simulink model "s_b16a4x512f"  (R2016b)
settings: Solver=VariableStepDiscrete  StartTime=0.0  StopTime=1  RelTol=1e-3
undefined symbols (not defined in the file): fft_stages, n_bits_ants, n_bits_xengs
libraries: xbsIndex_r4 x23057, casper_library_misc x150, xbsReplacements_r4 x9, casper_library_delays x8, xps_library x3
(part 8 of 210)

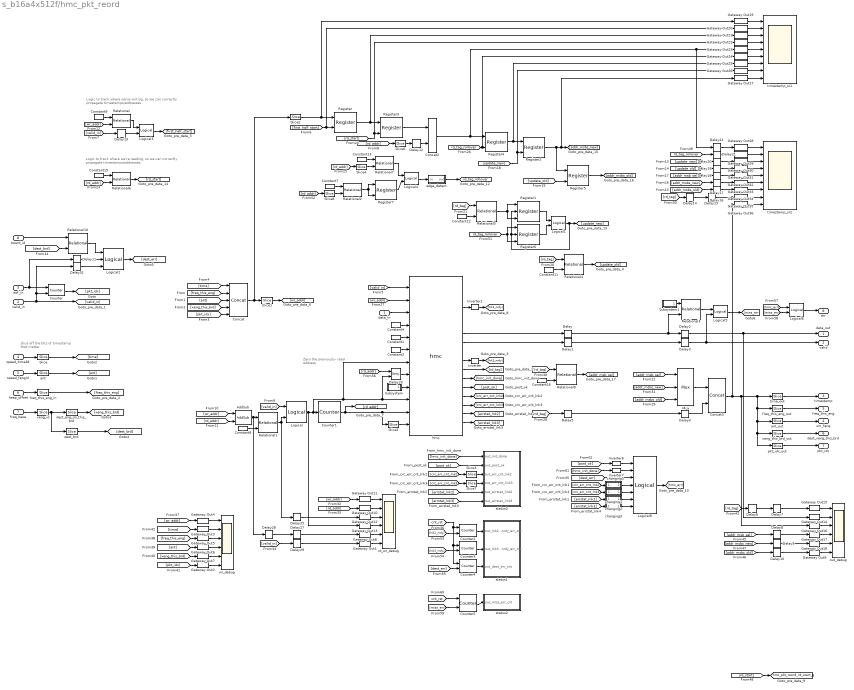
== system s_b16a4x512f/hmc_pkt_reord ==
  note: Zero the previously-
      | read address.
  note: Logic to track where we're writing,
      | so we can correctly propagate timestamps/addresses.
  note: slice off the bits of timestamp
      | that matter
  note: Logic to track where we're reading,
      | so we can correctly propagate timestamps/addresses.
  data_in : Inport
  valid_in : Inport  Port=2
  eof_in : Inport  Port=3
  spead_time48 : Inport  Port=4
  spead_fengid : Inport  Port=5
  heap_offset : Inport  Port=6
  freq_base : Inport  Port=7
  board_id : Inport  Port=8
  AddSub : xbsIndex_r4/AddSub  mode=Subtraction  use_carryin=off  use_carryout=off  en=off  latency=1  precision=User Defined  arith_type=Unsigned  n_bits=mem_depth  bin_pt=0  quantization=Truncate  overflow=Wrap  use_behavioral_HDL=off  hw_selection=Fabric  pipelined=off  dbl_ovrd=off  block_type=addsub
  Concat : xbsIndex_r4/Concat  num_inputs=5  dbl_ovrd=off  block_type=concat
  Concat2 : xbsIndex_r4/Concat  num_inputs=2  dbl_ovrd=off  block_type=concat
  Concat3 : xbsIndex_r4/Concat  num_inputs=2  dbl_ovrd=off  block_type=concat
  Constant1 : xbsIndex_r4/Constant  const=0  gui_display_data_type=Fixed-point  arith_type=Unsigned  n_bits=27  bin_pt=0  preci_type=Single  exp_width=8  frac_width=24  explicit_period=on  period=1  equ=P=C  opselect=C  inp2=PCIN>>17  opr=+  inp1=P  carry=CIN  dbl_ovrd=off  block_type=constant
  Constant11 : xbsIndex_r4/Constant  const=512*0.25  gui_display_data_type=Fixed-point  arith_type=Unsigned  n_bits=9  bin_pt=0  preci_type=Single  exp_width=8  frac_width=24  explicit_period=on  period=1  equ=P=C  opselect=C  inp2=PCIN>>17  opr=+  inp1=P  carry=CIN  dbl_ovrd=off  block_type=constant
  Constant12 : xbsIndex_r4/Constant  const=512*0.75  gui_display_data_type=Fixed-point  arith_type=Unsigned  n_bits=9  bin_pt=0  preci_type=Single  exp_width=8  frac_width=24  explicit_period=on  period=1  equ=P=C  opselect=C  inp2=PCIN>>17  opr=+  inp1=P  carry=CIN  dbl_ovrd=off  block_type=constant
  Constant13 : xbsIndex_r4/Constant  const=0  gui_display_data_type=Fixed-point  arith_type=Unsigned  n_bits=9  bin_pt=0  preci_type=Single  exp_width=8  frac_width=24  explicit_period=on  period=1  equ=P=C  opselect=C  inp2=PCIN>>17  opr=+  inp1=P  carry=CIN  dbl_ovrd=off  block_type=constant
  Constant15 : xbsIndex_r4/Constant  const=0  gui_display_data_type=Fixed-point  arith_type=Unsigned  n_bits=mem_depth  bin_pt=0  preci_type=Single  exp_width=8  frac_width=24  explicit_period=on  period=1  equ=P=C  opselect=C  inp2=PCIN>>17  opr=+  inp1=P  carry=CIN  dbl_ovrd=off  block_type=constant
  Constant16 : xbsIndex_r4/Constant  const=512*0.5  gui_display_data_type=Fixed-point  arith_type=Unsigned  n_bits=9  bin_pt=0  preci_type=Single  exp_width=8  frac_width=24  explicit_period=on  period=1  equ=P=C  opselect=C  inp2=PCIN>>17  opr=+  inp1=P  carry=CIN  dbl_ovrd=off  block_type=constant
  Constant2 : xbsIndex_r4/Constant  const=0  gui_display_data_type=Fixed-point  arith_type=Unsigned  n_bits=9  bin_pt=0  preci_type=Single  exp_width=8  frac_width=24  explicit_period=on  period=1  equ=P=C  opselect=C  inp2=PCIN>>17  opr=+  inp1=P  carry=CIN  dbl_ovrd=off  block_type=constant
  Constant4 : xbsIndex_r4/Constant  const=0  gui_display_data_type=Boolean  arith_type=Boolean  n_bits=64  bin_pt=0  preci_type=Single  exp_width=8  frac_width=24  explicit_period=on  period=1  equ=P=C  opselect=C  inp2=PCIN>>17  opr=+  inp1=P  carry=CIN  dbl_ovrd=off  block_type=constant
  Constant7 : xbsIndex_r4/Constant  const=511  gui_display_data_type=Fixed-point  arith_type=Unsigned  n_bits=9  bin_pt=0  preci_type=Single  exp_width=8  frac_width=24  explicit_period=on  period=1  equ=P=C  opselect=C  inp2=PCIN>>17  opr=+  inp1=P  carry=CIN  dbl_ovrd=off  block_type=constant
  Constant8 : xbsIndex_r4/Constant  const=2^(mem_depth-1)  gui_display_data_type=Fixed-point  arith_type=Unsigned  n_bits=mem_depth  bin_pt=0  preci_type=Single  exp_width=8  frac_width=24  explicit_period=on  period=1  equ=P=C  opselect=C  inp2=PCIN>>17  opr=+  inp1=P  carry=CIN  dbl_ovrd=off  block_type=constant
  Constant9 : xbsIndex_r4/Constant  const=2^(mem_depth)*1/4  gui_display_data_type=Fixed-point  arith_type=Unsigned  n_bits=mem_depth  bin_pt=0  preci_type=Single  exp_width=8  frac_width=24  explicit_period=on  period=1  equ=P=C  opselect=C  inp2=PCIN>>17  opr=+  inp1=P  carry=CIN  dbl_ovrd=off  block_type=constant
  Counter : xbsIndex_r4/Counter  cnt_type=Free Running  cnt_to=Inf  operation=Up  start_count=0  cnt_by_val=1  arith_type=Unsigned  n_bits=acc_bits-time_bits  bin_pt=0  load_pin=off  rst=on  en=on  explicit_period=on  period=1  use_behavioral_HDL=off  implementation=Fabric  dbl_ovrd=off  block_type=counter
  Counter1 : xbsIndex_r4/Counter  cnt_type=Free Running  cnt_to=Inf  operation=Up  start_count=0  cnt_by_val=1  arith_type=Unsigned  n_bits=mem_depth  bin_pt=0  load_pin=off  rst=off  en=on  explicit_period=on  period=1  use_behavioral_HDL=off  implementation=Fabric  dbl_ovrd=off  block_type=counter
  Counter2 : xbsIndex_r4/Counter  cnt_type=Free Running  cnt_to=Inf  operation=Up  start_count=0  cnt_by_val=1  arith_type=Unsigned  n_bits=8  bin_pt=0  load_pin=off  rst=on  en=on  explicit_period=on  period=1  use_behavioral_HDL=off  implementation=Fabric  dbl_ovrd=off  block_type=counter
  Counter3 : xbsIndex_r4/Counter  cnt_type=Free Running  cnt_to=Inf  operation=Up  start_count=0  cnt_by_val=1  arith_type=Unsigned  n_bits=8  bin_pt=0  load_pin=off  rst=on  en=on  explicit_period=on  period=1  use_behavioral_HDL=off  implementation=Fabric  dbl_ovrd=off  block_type=counter
  Counter4 : xbsIndex_r4/Counter  cnt_type=Free Running  cnt_to=Inf  operation=Up  start_count=0  cnt_by_val=1  arith_type=Unsigned  n_bits=16  bin_pt=0  load_pin=off  rst=on  en=on  explicit_period=on  period=1  use_behavioral_HDL=off  implementation=Fabric  dbl_ovrd=off  block_type=counter
  Counter5 : xbsIndex_r4/Counter  cnt_type=Free Running  cnt_to=Inf  operation=Up  start_count=0  cnt_by_val=1  arith_type=Unsigned  n_bits=32  bin_pt=0  load_pin=off  rst=on  en=on  explicit_period=on  period=1  use_behavioral_HDL=off  implementation=Fabric  dbl_ovrd=off  block_type=counter
  Delay{,1..10,12..22,25,27..29} (26 alike) : xbsIndex_r4/Delay  rst=off  infoeditControl=Selection of Reset will increase slice count due to use of real FFs and instead of SRLs  en=off  latency=1  reg_retiming=on  dbl_ovrd=off  block_type=delay
      settings: infoedit=Hardware notes: A delay line is a chain, each link of which is an SRL16 or SRL32 followed by a flip-flop.
  Delay11 : xbsIndex_r4/Delay  rst=off  infoeditControl=Selection of Reset will increase slice count due to use of real FFs and instead of SRLs  en=off  latency=2  reg_retiming=on  dbl_ovrd=off  block_type=delay
      settings: infoedit=Hardware notes: A delay line is a chain, each link of which is an SRL16 or SRL32 followed by a flip-flop.
  Delay23 : xbsIndex_r4/Delay  rst=off  infoeditControl=Selection of Reset will increase slice count due to use of real FFs and instead of SRLs  en=on  latency=62  reg_retiming=off  dbl_ovrd=off  block_type=delay
      settings: infoedit=Hardware notes: A delay line is a chain, each link of which is an SRL16 or SRL32 followed by a flip-flop.
  Delay31 : xbsIndex_r4/Delay  rst=off  infoeditControl=Selection of Reset will increase slice count due to use of real FFs and instead of SRLs  en=off  latency=2  reg_retiming=on  dbl_ovrd=off  block_type=delay
      settings: infoedit=Hardware notes: A delay line is a chain, each link of which is an SRL16 or SRL32 followed by a flip-flop.
  Gateway Out{1..18} (18 alike) : xbsIndex_r4/Gateway Out  inherit_from_input=off  hdl_port=off  rows=1  columns=1  UseAsDAC=off  DACChannel='1'  interface=None  automatic_assignment=on  address_offset=hex2dec('00')  intf_name=''  intf_description=''  timing_constraint=None  locs_specified=off  LOCs={}  io_standard={}  block_type=gatewayout
      settings: infoedit="Gateway out block.  Converts Xilinx fixed point inputs into ouputs of type Simulink integer, double, or fixed point.<P><P>Hardware notes:  In hardware these blocks become top level output ports or are discarded, depending on how they are configured."  xl_area=[0, 0, 0, 0, 0, 0, 0]  block_version=10.1.3
  Gateway Out{19..36} (18 alike) : xbsIndex_r4/Gateway Out  inherit_from_input=off  hdl_port=on  rows=1  columns=1  UseAsDAC=off  DACChannel='1'  interface=None  automatic_assignment=on  address_offset=hex2dec('00')  intf_name=''  intf_description=''  timing_constraint=None  locs_specified=off  LOCs={}  io_standard={}  block_type=gatewayout
  Inverter{,1,6..7} (4 alike) : xbsIndex_r4/Inverter  en=off  latency=0  dbl_ovrd=off  block_type=inv
  Logical : xbsIndex_r4/Logical  logical_function=AND  inputs=2  en=off  latency=1  precision=Full  arith_type=Unsigned  n_bits=16  bin_pt=0  align_bp=on  dbl_ovrd=off  block_type=logical
  Logical{1,3..5} (4 alike) : xbsIndex_r4/Logical  logical_function=AND  inputs=2  en=off  latency=0  precision=Full  arith_type=Unsigned  n_bits=16  bin_pt=0  align_bp=on  dbl_ovrd=off  block_type=logical
  Logical2 : xbsIndex_r4/Logical  logical_function=AND  inputs=3  en=off  latency=1  precision=Full  arith_type=Unsigned  n_bits=16  bin_pt=0  align_bp=on  dbl_ovrd=off  block_type=logical
  Logical6 : xbsIndex_r4/Logical  logical_function=OR  inputs=2  en=off  latency=0  precision=Full  arith_type=Unsigned  n_bits=16  bin_pt=0  align_bp=on  dbl_ovrd=off  block_type=logical
  Logical9 : xbsIndex_r4/Logical  logical_function=OR  inputs=7  en=off  latency=1  precision=Full  arith_type=Unsigned  n_bits=16  bin_pt=0  align_bp=on  dbl_ovrd=off  block_type=logical
  Mux : xbsIndex_r4/Mux  inputs=2  en=off  latency=1  precision=Full  arith_type=Unsigned  n_bits=16  bin_pt=14  quantization=Truncate  overflow=Wrap  dbl_ovrd=off  block_type=mux
  Register{,2..5,7} (6 alike) : xbsIndex_r4/Register  init=0  rst=off  en=on  dbl_ovrd=off  block_type=register
  Register1 : xbsIndex_r4/Register  init=0  rst=on  en=on  dbl_ovrd=off  block_type=register
  Register6 : xbsIndex_r4/Register  init=0  rst=on  en=on  dbl_ovrd=off  block_type=register
  Relational : xbsIndex_r4/Relational  mode=a>=b  op_type=Bool  en=off  latency=1  dbl_ovrd=off  block_type=relational
  Relational1 : xbsIndex_r4/Relational  mode=a>=b  op_type=Bool  en=off  latency=1  dbl_ovrd=off  block_type=relational
  Relational10 : xbsIndex_r4/Relational  mode=a!=b  op_type=Bool  en=off  latency=2  dbl_ovrd=off  block_type=relational
  Relational{2..3,6..7} (4 alike) : xbsIndex_r4/Relational  mode=a=b  op_type=Bool  en=off  latency=1  dbl_ovrd=off  block_type=relational
  Relational4 : xbsIndex_r4/Relational  mode=a=b  op_type=Bool  en=off  latency=0  dbl_ovrd=off  block_type=relational
  Relational5 : xbsIndex_r4/Relational  mode=a=b  op_type=Bool  en=off  latency=0  dbl_ovrd=off  block_type=relational
  Relational9 : xbsIndex_r4/Relational  mode=a>b  op_type=Bool  en=off  latency=1  dbl_ovrd=off  block_type=relational
  Slice : xbsIndex_r4/Slice  nbits=1  boolean_output=off  mode=Two Bit Locations  bit1=0  base1=MSB of Input  bit0=(freq_bits+1) + acc_bits  base0=LSB of Input  dbl_ovrd=off  block_type=slice
  Slice1 : xbsIndex_r4/Slice  nbits=mem_depth  boolean_output=off  mode=Lower Bit Location + Width  bit1=0  base1=MSB of Input  bit0=0  base0=LSB of Input  dbl_ovrd=off  block_type=slice
  Slice2 : xbsIndex_r4/Slice  nbits=27  boolean_output=off  mode=Two Bit Locations  bit1=0  base1=MSB of Input  bit0=mem_depth  base0=LSB of Input  dbl_ovrd=off  block_type=slice
  Slice3 : xbsIndex_r4/Slice  nbits=8  boolean_output=off  mode=Lower Bit Location + Width  bit1=0  base1=MSB of Input  bit0=0  base0=LSB of Input  dbl_ovrd=off  block_type=slice
  Slice4 : xbsIndex_r4/Slice  nbits=9  boolean_output=off  mode=Lower Bit Location + Width  bit1=0  base1=MSB of Input  bit0=0  base0=LSB of Input  dbl_ovrd=off  block_type=slice
  Slice5 : xbsIndex_r4/Slice  nbits=9  boolean_output=off  mode=Lower Bit Location + Width  bit1=0  base1=MSB of Input  bit0=0  base0=LSB of Input  dbl_ovrd=off  block_type=slice
  Slice6 : xbsIndex_r4/Slice  nbits=mem_depth  boolean_output=off  mode=Two Bit Locations  bit1=0  base1=MSB of Input  bit0=9  base0=LSB of Input  dbl_ovrd=off  block_type=slice
  Slice7 : xbsIndex_r4/Slice  nbits=8  boolean_output=off  mode=Lower Bit Location + Width  bit1=0  base1=MSB of Input  bit0=0  base0=LSB of Input  dbl_ovrd=off  block_type=slice
  Slice8 : xbsIndex_r4/Slice  nbits=9  boolean_output=off  mode=Lower Bit Location + Width  bit1=0  base1=MSB of Input  bit0=0  base0=LSB of Input  dbl_ovrd=off  block_type=slice
  Subsystem : Subsystem
  Subsystem1 : Subsystem
  ant : xbsIndex_r4/Slice  nbits=ant_bits  boolean_output=off  mode=Lower Bit Location + Width  bit1=0  base1=MSB of Input  bit0=0  base0=LSB of Input  dbl_ovrd=off  block_type=slice
      settings: block_version=10.1.3
  ant_out : xbsIndex_r4/Slice  nbits=ant_bits  boolean_output=off  mode=Lower Bit Location + Width  bit1=0  base1=MSB of Input  bit0=acc_bits+share_bits-time_bits  base0=LSB of Input  dbl_ovrd=off  block_type=slice
      settings: block_version=10.1.3
  changing0 : Subsystem
  changing1 : Subsystem
  changing2 : Subsystem
  changing3 : Subsystem
  dest_brd : xbsIndex_r4/Slice  nbits=xeng_bits-share_bits  boolean_output=off  mode=Upper Bit Location + Width  bit1=0  base1=MSB of Input  bit0=freq_bits-xeng_bits  base0=LSB of Input  dbl_ovrd=off  block_type=slice
      settings: block_version=10.1.3
  dest_eng_on_this_brd : xbsIndex_r4/Slice  nbits=share_bits  boolean_output=off  mode=Lower Bit Location + Width  bit1=0  base1=MSB of Input  bit0=0  base0=LSB of Input  dbl_ovrd=off  block_type=slice
      settings: block_version=10.1.3
  edge_detect : Subsystem  AncestorBlock=casper_library_misc/edge_detect  mask(edge_detect){edge=Falling, polarity=Active High, x_in=[0 0.08 0.08 0.16 0.16 0.24 0.24 0.32 0.32 0.4], y_in=[-1 -1  1  1  1  1  1  1  1  1], x_out=[0.6 0.68 0.68 0.76 0.76 0.84 0.84 0.92 0.92 1], y_out=[-1 -1  1  1 -1 -1 -1 -1 -1 -1]}
      mask prompts: edge "Edge Type"; polarity "Output Polarity"; x_in "Input X Positions"; y_in "Input Y Positions"; x_out "Output X Positions"; y_out "Output Y Positions"
      mask help: Output is active for one-cycle after each edge of the specified type (i.e. rising, falling or both).
      mask init: same as s_b16a4x512f/edge_detect
      settings: AttributesFormatString=|
      | falling edges
      | active high
      mask Help: Output is active for one-cycle after each edge of the specified type (i.e. rising, falling, or both).  Latency is zero.
      mask TypeOptions edge: Rising | Falling | Both
      mask TypeOptions polarity: Active High | Active Low
      mask Display:
      | plot(x_in_num,0.5+y_in_num*0.2);
      | plot(x_out_num,0.5+y_out_num*0.2);
  freq_this_eng_in : xbsIndex_r4/Slice  nbits=freq_bits - xeng_bits  boolean_output=off  mode=Lower Bit Location + Width  bit1=0  base1=LSB of Input  bit0=acc_bits-1+3  base0=LSB of Input  dbl_ovrd=off  block_type=slice
      settings: block_version=10.1.3
  freq_this_eng_out : xbsIndex_r4/Slice  nbits=freq_bits - xeng_bits  boolean_output=off  mode=Lower Bit Location + Width  bit1=0  base1=LSB of Input  bit0=acc_bits+share_bits+ant_bits-time_bits  base0=LSB of Input  dbl_ovrd=off  block_type=slice
      settings: block_version=10.1.3
  hmc : xps_library/hmc  Tag=xps:hmc  mez=2  sim_depth=12  sim_latency=10  sim_rand=on
      link override sim_mem1: randread=off
      link override sim_mem2/sfunc: depth_bits=12
  out_debug : Scope  NumInputPorts=6
  pkt_idx_out : xbsIndex_r4/Slice  nbits=acc_bits-time_bits  boolean_output=off  mode=Lower Bit Location + Width  bit1=freq_bits  base1=LSB of Input  bit0=0  base0=LSB of Input  dbl_ovrd=off  block_type=slice
      settings: block_version=10.1.3
  rd_wr_debug : Scope  NumInputPorts=6
  status0 : Subsystem  Tag=xps:sw_reg  AncestorBlock=xps_library/software_register  mask(swreg){io_dir=To Processor, io_delay=0, sample_period=1, names=[init_done post_ok err_cnt_lnk2 err_cnt_link3 errstat_link2 errstat_link3], bitwidths=[1 1 8 8 7 7], bin_pts=0, arith_types=[2 2 0 0 0 0], sim_port=off, show_format=on}
      mask prompts: io_dir "I/O direction"; io_delay "I/O delay"; sample_period "Sample period"; names "Bitfield names [msb...lsb]"; bitwidths "Bitfield widths"; bin_pts "Bitfield binary pts"; arith_types "Bitfield types, ufix=0, fix=1, bool=2"; sim_port "Provide sim input/output?"; show_format "Print format string?"
      mask help: A 32-bit software-accessible register. Can be divided into bitfields of varying widths and types using the fields in the block mask.
      mask init:
      | swreg_init(gcb)
      settings: AttributesFormatString=6 outputs:b,b,uf8.0,uf8.0,uf7.0,uf7.0 = 32 bits
      mask TypeOptions io_dir: To Processor | From Processor
      mask Callback io_dir:
      | mask_enables = get_param(gcb, 'MaskEnables');
      | mask_names = get_param(gcb, 'MaskNames');
      | if strcmp(get_param(gcb, 'io_dir'), 'To Processor'),
      |     mask_enables{ismember(mask_names, 'sample_period')} = 'off';
      | else
      |     mask_enables{ismember(mask_names, 'sample_period')} = 'on';
      | end
      | set_param(gcb, 'MaskEnables', mask_enables);
  status1 : Subsystem  Tag=xps:sw_reg  AncestorBlock=xps_library/software_register  mask(swreg){io_dir=To Processor, io_delay=0, sample_period=1, names=[lnk2_nrdy_err_cnt lnk3_nrdy_err_cnt dest_err_cnt], bitwidths=[8 8 16], bin_pts=0, arith_types=0, sim_port=off, show_format=on}
      mask prompts: io_dir "I/O direction"; io_delay "I/O delay"; sample_period "Sample period"; names "Bitfield names [msb...lsb]"; bitwidths "Bitfield widths"; bin_pts "Bitfield binary pts"; arith_types "Bitfield types, ufix=0, fix=1, bool=2"; sim_port "Provide sim input/output?"; show_format "Print format string?"
      mask help: A 32-bit software-accessible register. Can be divided into bitfields of varying widths and types using the fields in the block mask.
      mask init:
      | swreg_init(gcb)
      settings: AttributesFormatString=3 outputs:uf8.0,uf8.0,uf16.0 = 32 bits
      mask TypeOptions io_dir: To Processor | From Processor
      mask Callback io_dir:
      | mask_enables = get_param(gcb, 'MaskEnables');
      | mask_names = get_param(gcb, 'MaskNames');
      | if strcmp(get_param(gcb, 'io_dir'), 'To Processor'),
      |     mask_enables{ismember(mask_names, 'sample_period')} = 'off';
      | else
      |     mask_enables{ismember(mask_names, 'sample_period')} = 'on';
      | end
      | set_param(gcb, 'MaskEnables', mask_enables);
  status2 : Subsystem  Tag=xps:sw_reg  AncestorBlock=xps_library/software_register  mask(swreg){io_dir=To Processor, io_delay=0, sample_period=1, names=[miss_err_cnt], bitwidths=[32], bin_pts=0, arith_types=0, sim_port=off, show_format=on}
      mask prompts: io_dir "I/O direction"; io_delay "I/O delay"; sample_period "Sample period"; names "Bitfield names [msb...lsb]"; bitwidths "Bitfield widths"; bin_pts "Bitfield binary pts"; arith_types "Bitfield types, ufix=0, fix=1, bool=2"; sim_port "Provide sim input/output?"; show_format "Print format string?"
      mask help: A 32-bit software-accessible register. Can be divided into bitfields of varying widths and types using the fields in the block mask.
      mask init:
      | swreg_init(gcb)
      settings: AttributesFormatString=1output:uf32.0 = 32 bits
      mask TypeOptions io_dir: To Processor | From Processor
      mask Callback io_dir:
      | mask_enables = get_param(gcb, 'MaskEnables');
      | mask_names = get_param(gcb, 'MaskNames');
      | if strcmp(get_param(gcb, 'io_dir'), 'To Processor'),
      |     mask_enables{ismember(mask_names, 'sample_period')} = 'off';
      | else
      |     mask_enables{ismember(mask_names, 'sample_period')} = 'on';
      | end
      | set_param(gcb, 'MaskEnables', mask_enables);
  time_out : xbsIndex_r4/Slice  nbits=1  boolean_output=off  mode=Two Bit Locations  bit1=0  base1=MSB of Input  bit0=acc_bits+share_bits+ant_bits+freq_bits-xeng_bits-time_bits  base0=LSB of Input  dbl_ovrd=off  block_type=slice
  timestamp_sr1 : Scope  NumInputPorts=9
  timestamp_sr2 : Scope  NumInputPorts=9
  wr_debug : Scope  NumInputPorts=6
  xeng_id : xbsIndex_r4/Slice  nbits=xeng_bits  boolean_output=off  mode=Lower Bit Location + Width  bit1=freq_bits  base1=LSB of Input  bit0=freq_bits-xeng_bits  base0=LSB of Input  dbl_ovrd=off  block_type=slice
      settings: block_version=10.1.3
  xeng_this_brd_out : xbsIndex_r4/Slice  nbits=share_bits  boolean_output=off  mode=Lower Bit Location + Width  bit1=freq_bits  base1=LSB of Input  bit0=acc_bits-time_bits  base0=LSB of Input  dbl_ovrd=off  block_type=slice
      settings: block_version=10.1.3
  data_out : Outport
  valid : Outport  Port=2
  timestamp : Outport  Port=3
  src_feng : Outport  Port=4
  freq_this_eng : Outport  Port=5
  dest_xeng_this_brd : Outport  Port=6
  pkt_idx : Outport  Port=7
  err : Outport  Port=8
  tag scope: hmc_pkt_reord_rd_start_g=global, rd_tag_rollover=global
  wires:
  Gateway Out1/1 -> rd_wr_debug/6
  Gateway Out10/1 -> rd_wr_debug/2
  Gateway Out11/1 -> rd_wr_debug/1
  Gateway Out12/1 -> rd_wr_debug/3
  Gateway Out13/1 -> rd_wr_debug/4
  Gateway Out8/1 -> rd_wr_debug/5
  heap_offset/1 -> freq_this_eng_in/1
  xeng_id/1 -> dest_eng_on_this_brd/1, dest_brd/1
  spead_fengid/1 -> ant/1
  spead_time48/1 -> Slice/1
  freq_base/1 -> xeng_id/1
  [xeng_this_brd] -> Concat/4
  [pkt_idx] -> Concat/5
  [freq_this_eng] -> Concat/2
  [ant] -> Concat/3
  [time] -> Concat/1
  Concat/1 -> Slice2/1, Slice1/1
  data_in/1 -> hmc/3
  eof_in/1 -> Counter/1, Delay11/1
  valid_in/1 -> [valid_in], Delay31/1, Counter/2
  [valid_in] -> hmc/1
  Counter/1 -> [pkt_idx]
  ant/1 -> [ant]
  Slice/1 -> [time]
  dest_eng_on_this_brd/1 -> [xeng_this_brd]
  freq_this_eng_in/1 -> [freq_this_eng]
  Delay23/1 -> hmc/8
  Subsystem/1(Out1) -> hmc/9
  [first_half_start] -> Gateway Out20/1, Register/2
  Slice2/1 -> Gateway Out19/1, Register/1
  Counter1/1 -> hmc/11, Slice5/1, [rd_addr]
  Slice5/1 -> hmc/12
  [valid_in] -> Logical/1
  Constant8/1 -> Relational1/2
  AddSub/1 -> Delay28/1, Relational1/1
  [wr_addr] -> AddSub/1
  [rd_addr] -> AddSub/2
  Relational1/1 -> Delay25/1, Logical/2
  Constant9/1 -> Relational/1
  [wr_addr] -> Relational/2
  [rd_tag] -> Relational4/1
  Constant11/1 -> Relational4/2
  Constant12/1 -> Relational5/2
  [rd_tag] -> Relational5/1
  Constant15/1 -> Relational6/1
  [rd_addr] -> Relational6/2
  Relational6/1 -> [rd_start]
  Register/1 -> Gateway Out21/1, Register3/1
  [rd_start] -> Gateway Out22/1, Register3/2
  Constant13/1 -> Relational7/1
  [rd_addr] -> Slice4/1
  Slice4/1 -> Relational7/2
  Slice1/1 -> [wr_addr]
  [wr_addr] -> hmc/2
  [rd_tag_rollover] -> Gateway Out24/1, Register4/2
  Register3/1 -> Concat2/1
  Slice6/1 -> Delay12/1
  [rd_addr] -> Slice6/1
  Concat2/1 -> Gateway Out23/1, Delay22/1, Register4/1
  Relational4/1 -> [update_old]
  [rd_tag] -> Delay5/1
  Register4/1 -> Gateway Out25/1, Register2/1
  Register2/1 -> Gateway Out27/1, [addr_msbs_new], Register5/1
  [update_old] -> Register5/2
  Register5/1 -> [addr_msbs_old]
  Constant16/1 -> Relational9/2
  [rd_tag] -> Relational9/1
  Relational9/1 -> [addr_msb_sel]
  Mux/1 -> Concat3/1
  [addr_msb_sel] -> Mux/1
  [addr_msbs_old] -> Mux/3
  [addr_msbs_new] -> Mux/2
  Concat3/1 -> Gateway Out36/1, Gateway Out16/1, pkt_idx_out/1, xeng_this_brd_out/1, ant_out/1, freq_this_eng_out/1, time_out/1
  time_out/1 -> timestamp/1
  freq_this_eng_out/1 -> freq_this_eng/1
  ant_out/1 -> src_feng/1
  xeng_this_brd_out/1 -> dest_xeng_this_brd/1
  pkt_idx_out/1 -> pkt_idx/1
  Delay/1 -> Relational3/2, Delay2/1
  Delay1/1 -> Delay3/1
  Delay2/1 -> data_out/1, Gateway Out14/1
  Delay4/1 -> Concat3/2
  Delay5/1 -> Delay4/1
  [wr_addr] -> Gateway Out11/1
  [rd_addr] -> Gateway Out10/1
  dest_brd/1 -> [dest_brd]
  Gateway Out2/1 -> wr_debug/6
  Gateway Out3/1 -> wr_debug/2
  Gateway Out4/1 -> wr_debug/1
  Gateway Out5/1 -> wr_debug/3
  Gateway Out6/1 -> wr_debug/4
  Gateway Out7/1 -> wr_debug/5
  [wr_addr] -> Gateway Out4/1
  [time] -> Gateway Out3/1
  [freq_this_eng] -> Gateway Out5/1
  [ant] -> Gateway Out6/1
  [xeng_this_brd] -> Gateway Out7/1
  [pkt_idx] -> Gateway Out2/1
  Gateway Out9/1 -> out_debug/6
  Gateway Out14/1 -> out_debug/2
  Gateway Out15/1 -> out_debug/1
  Gateway Out16/1 -> out_debug/3
  Gateway Out17/1 -> out_debug/4
  Gateway Out18/1 -> out_debug/5
  [addr_msb_sel] -> Delay8/1
  [addr_msbs_new] -> Delay9/1
  [addr_msbs_old] -> Delay10/1
  [rd_tag] -> Delay6/1
  Delay6/1 -> Delay7/1
  Delay7/1 -> Gateway Out15/1
  Delay8/1 -> Gateway Out17/1
  Delay9/1 -> Gateway Out18/1
  Delay10/1 -> Gateway Out9/1
  Slice3/1 -> status0/3(out_err_cnt_lnk2)
  Slice7/1 -> status0/4(out_err_cnt_link3)
  [dest_brd] -> Relational10/2
  board_id/1 -> Relational10/1
  Relational10/1 -> Logical2/1
  Delay11/1 -> Logical2/2
  Gateway Out23/1 -> timestamp_sr1/5
  Gateway Out26/1 -> timestamp_sr1/8
  Gateway Out20/1 -> timestamp_sr1/2
  Gateway Out19/1 -> timestamp_sr1/1
  Gateway Out25/1 -> timestamp_sr1/7
  Gateway Out22/1 -> timestamp_sr1/4
  Gateway Out21/1 -> timestamp_sr1/3
  Gateway Out24/1 -> timestamp_sr1/6
  Gateway Out27/1 -> timestamp_sr1/9
  [update_new] -> Gateway Out26/1, Register2/2
  Delay12/1 -> Concat2/2
  Logical3/1 -> [first_half_start]
  Relational/1 -> Logical3/1
  [valid_in] -> Delay13/1
  Delay13/1 -> Logical3/2
  Gateway Out32/1 -> timestamp_sr2/5
  Gateway Out35/1 -> timestamp_sr2/8
  Gateway Out29/1 -> timestamp_sr2/2
  Gateway Out28/1 -> timestamp_sr2/1
  Gateway Out34/1 -> timestamp_sr2/7
  Gateway Out31/1 -> timestamp_sr2/4
  Gateway Out30/1 -> timestamp_sr2/3
  Gateway Out33/1 -> timestamp_sr2/6
  Gateway Out36/1 -> timestamp_sr2/9
  [rd_tag_rollover] -> Delay21/1
  [update_new] -> Delay20/1
  [update_old] -> Delay19/1
  [addr_msb_sel] -> Delay18/1
  [addr_msbs_new] -> Delay17/1
  [addr_msbs_old] -> Delay16/1
  [rd_tag] -> Delay14/1
  Delay14/1 -> Delay15/1
  Delay15/1 -> Gateway Out35/1
  Delay16/1 -> Gateway Out34/1
  Delay17/1 -> Gateway Out33/1
  Delay18/1 -> Gateway Out32/1
  Delay19/1 -> Gateway Out31/1
  Delay20/1 -> Gateway Out30/1
  Delay21/1 -> Gateway Out29/1
  Delay22/1 -> Gateway Out28/1
  Relational5/1 -> Register1/3, Register1/1
  [rd_tag_rollover] -> Register6/1, Register6/3
  Register1/1 -> Logical1/1
  Register6/1 -> Logical1/2
  Logical1/1 -> Register6/2, Register1/2, [update_new]
  Relational7/1 -> Logical4/1
  Register7/1 -> Logical4/2
  Constant7/1 -> Relational2/1
  [rd_addr] -> Slice8/1
  Slice8/1 -> Relational2/2
  Relational2/1 -> Register7/2, Register7/1
  Logical4/1 -> edge_detect/1(in)
  edge_detect/1(out) -> [rd_tag_rollover]
  [valid_in] -> Delay29/1
  Delay25/1 -> Gateway Out12/1
  Delay27/1 -> Gateway Out8/1
  Delay28/1 -> Delay27/1
  Delay29/1 -> Gateway Out1/1
  Subsystem1/1(Out1) -> Relational3/1
  Relational3/1 -> Logical5/1
  Delay3/1 -> Logical5/2, valid/1
  Logical2/1 -> [dest_err]
  Logical6/1 -> err/1
  [cnt_rst] -> Counter4/1, Counter3/1, Counter2/1
  Counter2/1 -> status1/1(out_lnk2_nrdy_err_cnt)
  Counter3/1 -> status1/2(out_lnk3_nrdy_err_cnt)
  Counter4/1 -> status1/3(out_dest_err_cnt)
  hmc/9 -> Inverter/1
  Inverter/1 -> [lnk3_nrdy]
  hmc/3 -> Inverter1/1
  Inverter1/1 -> [lnk2_nrdy]
  [dest_err] -> Counter4/2
  [lnk2_nrdy] -> Counter2/2
  [lnk3_nrdy] -> Counter3/2
  Logical/1 -> Gateway Out13/1, Delay23/2, hmc/10, hmc/7, Counter1/1
  Delay31/1 -> Logical2/3
  [rd_start] -> [hmc_pkt_reord_rd_start_g]
  Constant2/1 -> hmc/6
  Constant1/1 -> hmc/5
  Constant4/1 -> hmc/4
  hmc/10 -> [rd_tag]
  hmc/6 -> Delay/1
  hmc/7 -> Delay1/1
  [post_ok] -> Inverter6/1
  Inverter6/1 -> Logical9/1
  [hmc_init_done] -> Inverter7/1
  hmc/11 -> [hmc_init_done]
  hmc/12 -> [post_ok]
  hmc/13 -> [crc_err_cnt_lnk2]
  hmc/14 -> [crc_err_cnt_lnk3]
  hmc/15 -> [errstat_lnk2]
  hmc/16 -> [errstat_lnk3]
  [post_ok] -> status0/2(out_post_ok)
  [hmc_init_done] -> status0/1(out_init_done)
  [crc_err_cnt_lnk2] -> Slice3/1
  [crc_err_cnt_lnk3] -> Slice7/1
  [errstat_lnk2] -> status0/5(out_errstat_link2)
  [errstat_lnk3] -> status0/6(out_errstat_link3)
  Inverter7/1 -> Logical9/2
  [dest_err] -> Logical9/3
  [crc_err_cnt_lnk2] -> changing0/1(In1)
  changing0/1(Out1) -> Logical9/4
  changing3/1(Out1) -> Logical9/7
  changing1/1(Out1) -> Logical9/5
  changing2/1(Out1) -> Logical9/6
  [crc_err_cnt_lnk3] -> changing1/1(In1)
  [errstat_lnk2] -> changing2/1(In1)
  [errstat_lnk3] -> changing3/1(In1)
  Logical9/1 -> [hmc_err]
  [hmc_err] -> Logical6/1
  [rd_addr] -> Delay23/1
  [miss_err] -> Logical6/2
  Logical5/1 -> [miss_err]
  [miss_err] -> Counter5/2
  [cnt_rst] -> Counter5/1
  Counter5/1 -> status2/1(out_miss_err_cnt)

== system s_b16a4x512f/hmc_pkt_reord_status ==
  out_err_cnt : Inport
  assert_err_cnt : xbsIndex_r4/Assert  assert_type=on  type_source=Explicitly  gui_display_data_type=Fixed-point  arith_type=Unsigned  n_bits=32  bin_pt=0  preci_type=Single  exp_width=8  frac_width=24  assert_rate=off  rate_source=Explicitly  period=1  output_port=on  block_type=assert
  cast_gw : xbsIndex_r4/Convert  gui_display_data_type=Fixed-point  arith_type=Unsigned  n_bits=32  bin_pt=0  float_type=Single  exp_bits=8  fraction_bits=24  quantization=Truncate  overflow=Wrap  en=off  latency=1  pipeline=off  dbl_ovrd=off  block_type=convert
  io_delay : xbsIndex_r4/Delay  rst=off  infoeditControl=Selection of Reset will increase slice count due to use of real FFs and instead of SRLs  en=off  latency=0  reg_retiming=on  dbl_ovrd=off  block_type=delay
      settings: infoedit=Hardware notes: A delay line is a chain, each link of which is an SRL16 or SRL32 followed by a flip-flop.
  reint1 : xbsIndex_r4/Reinterpret  force_arith_type=on  arith_type=Unsigned  force_bin_pt=on  bin_pt=0  block_type=reinterpret
  s_b16a4x512f_hmc_pkt_reord_status_user_data_in : xbsIndex_r4/Gateway Out  inherit_from_input=off  hdl_port=on  rows=1  columns=1  UseAsDAC=off  DACChannel='1'  interface=None  automatic_assignment=on  address_offset=hex2dec('00')  intf_name=''  intf_description=''  timing_constraint=None  locs_specified=off  LOCs={}  io_standard={}  block_type=gatewayout
  sim_out : Terminator
  wires:
  io_delay/1 -> cast_gw/1
  cast_gw/1 -> s_b16a4x512f_hmc_pkt_reord_status_user_data_in/1
  s_b16a4x512f_hmc_pkt_reord_status_user_data_in/1 -> sim_out/1
  out_err_cnt/1 -> assert_err_cnt/1
  assert_err_cnt/1 -> reint1/1
  reint1/1 -> io_delay/1

== system s_b16a4x512f/miss_cnt0 ==
  Convert : xbsIndex_r4/Convert  gui_display_data_type=Fixed-point  arith_type=Unsigned  n_bits=6  bin_pt=0  float_type=Single  exp_bits=8  fraction_bits=24  quantization=Truncate  overflow=Wrap  en=off  latency=0  pipeline=off  dbl_ovrd=off  block_type=convert
  Counter1 : xbsIndex_r4/Counter  cnt_type=Free Running  cnt_to=1023  operation=Up  start_count=0  cnt_by_val=1  arith_type=Unsigned  n_bits=6  bin_pt=0  load_pin=off  rst=on  en=on  explicit_period=on  period=1  use_behavioral_HDL=on  implementation=Fabric  use_rpm=on  dbl_ovrd=off  block_type=counter
      settings: xl_area=[0, 0, 0, 0, 0, 0, 0]
  Delay1 : Subsystem  AncestorBlock=casper_library_delays/pipeline  mask(pipeline){latency=2}
      mask help:
      | An explicitly laid-out delay line to avoid mapping to SRL16s
      | for use in pipelining to help achieve timing closure.
      mask init:
      | pipeline_init(gcb,'latency',latency);
      settings: AttributesFormatString=Latency = %<latency>
      mask Display:
      | port_label('input', 1, 'd');
      | port_label('output', 1, 'q');
      | disp(['Z^-', num2str(latency)]);
  Delay11 : Subsystem  AncestorBlock=casper_library_delays/pipeline  mask(pipeline){latency=2}
      mask help:
      | An explicitly laid-out delay line to avoid mapping to SRL16s
      | for use in pipelining to help achieve timing closure.
      mask init:
      | pipeline_init(gcb,'latency',latency);
      settings: AttributesFormatString=Latency = %<latency>
      mask Display:
      | port_label('input', 1, 'd');
      | port_label('output', 1, 'q');
      | disp(['Z^-', num2str(latency)]);
  Delay15 : Subsystem  AncestorBlock=casper_library_delays/pipeline  mask(pipeline){latency=2}
      mask help:
      | An explicitly laid-out delay line to avoid mapping to SRL16s
      | for use in pipelining to help achieve timing closure.
      mask init:
      | pipeline_init(gcb,'latency',latency);
      settings: AttributesFormatString=Latency = %<latency>
      mask Display:
      | port_label('input', 1, 'd');
      | port_label('output', 1, 'q');
      | disp(['Z^-', num2str(latency)]);
  Delay2 : Subsystem  AncestorBlock=casper_library_delays/pipeline  mask(pipeline){latency=2}
      mask help:
      | An explicitly laid-out delay line to avoid mapping to SRL16s
      | for use in pipelining to help achieve timing closure.
      mask init:
      | pipeline_init(gcb,'latency',latency);
      settings: AttributesFormatString=Latency = %<latency>
      mask Display:
      | port_label('input', 1, 'd');
      | port_label('output', 1, 'q');
      | disp(['Z^-', num2str(latency)]);
  Delay3 : Subsystem  AncestorBlock=casper_library_delays/pipeline  mask(pipeline){latency=2}
      mask help:
      | An explicitly laid-out delay line to avoid mapping to SRL16s
      | for use in pipelining to help achieve timing closure.
      mask init:
      | pipeline_init(gcb,'latency',latency);
      settings: AttributesFormatString=Latency = %<latency>
      mask Display:
      | port_label('input', 1, 'd');
      | port_label('output', 1, 'q');
      | disp(['Z^-', num2str(latency)]);
  Delay4 : Subsystem  AncestorBlock=casper_library_delays/pipeline  mask(pipeline){latency=1}
      mask help:
      | An explicitly laid-out delay line to avoid mapping to SRL16s
      | for use in pipelining to help achieve timing closure.
      mask init:
      | pipeline_init(gcb,'latency',latency);
      settings: AttributesFormatString=Latency = %<latency>
      mask Display:
      | port_label('input', 1, 'd');
      | port_label('output', 1, 'q');
      | disp(['Z^-', num2str(latency)]);
  Delay5 : Subsystem  AncestorBlock=casper_library_delays/pipeline  mask(pipeline){latency=2}
      mask help:
      | An explicitly laid-out delay line to avoid mapping to SRL16s
      | for use in pipelining to help achieve timing closure.
      mask init:
      | pipeline_init(gcb,'latency',latency);
      settings: AttributesFormatString=Latency = %<latency>
      mask Display:
      | port_label('input', 1, 'd');
      | port_label('output', 1, 'q');
      | disp(['Z^-', num2str(latency)]);
  Delay6 : Subsystem  AncestorBlock=casper_library_delays/pipeline  mask(pipeline){latency=3}
      mask help:
      | An explicitly laid-out delay line to avoid mapping to SRL16s
      | for use in pipelining to help achieve timing closure.
      mask init:
      | pipeline_init(gcb,'latency',latency);
      settings: AttributesFormatString=Latency = %<latency>
      mask Display:
      | port_label('input', 1, 'd');
      | port_label('output', 1, 'q');
      | disp(['Z^-', num2str(latency)]);
  Delay7 : Subsystem  AncestorBlock=casper_library_delays/pipeline  mask(pipeline){latency=2}
      mask help:
      | An explicitly laid-out delay line to avoid mapping to SRL16s
      | for use in pipelining to help achieve timing closure.
      mask init:
      | pipeline_init(gcb,'latency',latency);
      settings: AttributesFormatString=Latency = %<latency>
      mask Display:
      | port_label('input', 1, 'd');
      | port_label('output', 1, 'q');
      | disp(['Z^-', num2str(latency)]);
  Delay8 : Subsystem  AncestorBlock=casper_library_delays/pipeline  mask(pipeline){latency=2}
      mask help:
      | An explicitly laid-out delay line to avoid mapping to SRL16s
      | for use in pipelining to help achieve timing closure.
      mask init:
      | pipeline_init(gcb,'latency',latency);
      settings: AttributesFormatString=Latency = %<latency>
      mask Display:
      | port_label('input', 1, 'd');
      | port_label('output', 1, 'q');
      | disp(['Z^-', num2str(latency)]);
  Delay9 : Subsystem  AncestorBlock=casper_library_delays/pipeline  mask(pipeline){latency=2}
      mask help:
      | An explicitly laid-out delay line to avoid mapping to SRL16s
      | for use in pipelining to help achieve timing closure.
      mask init:
      | pipeline_init(gcb,'latency',latency);
      settings: AttributesFormatString=Latency = %<latency>
      mask Display:
      | port_label('input', 1, 'd');
      | port_label('output', 1, 'q');
      | disp(['Z^-', num2str(latency)]);
  Delay96 : Subsystem  AncestorBlock=casper_library_delays/pipeline  mask(pipeline){latency=2}
      mask help:
      | An explicitly laid-out delay line to avoid mapping to SRL16s
      | for use in pipelining to help achieve timing closure.
      mask init:
      | pipeline_init(gcb,'latency',latency);
      settings: AttributesFormatString=Latency = %<latency>
      mask Display:
      | port_label('input', 1, 'd');
      | port_label('output', 1, 'q');
      | disp(['Z^-', num2str(latency)]);
  Delay97 : Subsystem  AncestorBlock=casper_library_delays/pipeline  mask(pipeline){latency=2}
      mask help:
      | An explicitly laid-out delay line to avoid mapping to SRL16s
      | for use in pipelining to help achieve timing closure.
      mask init:
      | pipeline_init(gcb,'latency',latency);
      settings: AttributesFormatString=Latency = %<latency>
      mask Display:
      | port_label('input', 1, 'd');
      | port_label('output', 1, 'q');
      | disp(['Z^-', num2str(latency)]);
  Delay98 : Subsystem  AncestorBlock=casper_library_delays/pipeline  mask(pipeline){latency=2}
      mask help:
      | An explicitly laid-out delay line to avoid mapping to SRL16s
      | for use in pipelining to help achieve timing closure.
      mask init:
      | pipeline_init(gcb,'latency',latency);
      settings: AttributesFormatString=Latency = %<latency>
      mask Display:
      | port_label('input', 1, 'd');
      | port_label('output', 1, 'q');
      | disp(['Z^-', num2str(latency)]);
  Logical1 : xbsIndex_r4/Logical  logical_function=AND  inputs=2  en=off  latency=1  precision=Full  arith_type=Unsigned  n_bits=8  bin_pt=2  align_bp=on  dbl_ovrd=off  block_type=logical
      settings: xl_area=[0, 0, 0, 0, 0, 0, 0]
  Logical2 : xbsIndex_r4/Logical  logical_function=AND  inputs=2  en=off  latency=1  precision=Full  arith_type=Unsigned  n_bits=8  bin_pt=2  align_bp=on  dbl_ovrd=off  block_type=logical
      settings: xl_area=[0, 0, 0, 0, 0, 0, 0]
  Logical3 : xbsIndex_r4/Logical  logical_function=AND  inputs=2  en=off  latency=1  precision=Full  arith_type=Unsigned  n_bits=8  bin_pt=2  align_bp=on  dbl_ovrd=off  block_type=logical
      settings: xl_area=[0, 0, 0, 0, 0, 0, 0]
  Register : xbsIndex_r4/Register  init=0  rst=on  en=on  dbl_ovrd=off  block_type=register
  Slice : xbsIndex_r4/Slice  nbits=16  boolean_output=off  mode=Two Bit Locations  bit1=0  base1=MSB of Input  bit0=xeng_int_bits  base0=LSB of Input  dbl_ovrd=off  block_type=slice
      settings: infoedit="Extracts a given range of bits from each input sample and presents it at the output.  The output type is ordinarily unsigned with binary point at zero, but can be Boolean when the slice is one bit wide.<P><P>Hardware notes: In hardware this block costs nothing."  block_version=10.1.3
  ant_cnt : xbsIndex_r4/Counter  cnt_type=Free Running  cnt_to=1023  operation=Up  start_count=0  cnt_by_val=1  arith_type=Unsigned  n_bits=xeng_int_bits + n_ants_bits  bin_pt=0  load_pin=off  rst=on  en=on  explicit_period=on  period=1  use_behavioral_HDL=on  implementation=Fabric  use_rpm=on  dbl_ovrd=off  block_type=counter
      settings: xl_area=[0, 0, 0, 0, 0, 0, 0]
  sync_ctr1 : xbsIndex_r4/Counter  cnt_type=Free Running  cnt_to=1023  operation=Up  start_count=0  cnt_by_val=1  arith_type=Unsigned  n_bits=6  bin_pt=0  load_pin=off  rst=on  en=on  explicit_period=on  period=1  use_behavioral_HDL=off  implementation=Fabric  use_rpm=on  dbl_ovrd=off  block_type=counter
      settings: xl_area=[0, 0, 0, 0, 0, 0, 0]
  sync_ctr5 : xbsIndex_r4/Counter  cnt_type=Free Running  cnt_to=1023  operation=Up  start_count=0  cnt_by_val=1  arith_type=Unsigned  n_bits=6  bin_pt=0  load_pin=off  rst=on  en=on  explicit_period=on  period=1  use_behavioral_HDL=on  implementation=Fabric  use_rpm=on  dbl_ovrd=off  block_type=counter
      settings: xl_area=[0, 0, 0, 0, 0, 0, 0]
  sync_ctr6 : xbsIndex_r4/Counter  cnt_type=Free Running  cnt_to=1023  operation=Up  start_count=0  cnt_by_val=1  arith_type=Unsigned  n_bits=6  bin_pt=0  load_pin=off  rst=on  en=on  explicit_period=on  period=1  use_behavioral_HDL=on  implementation=Fabric  use_rpm=on  dbl_ovrd=off  block_type=counter
      settings: xl_area=[0, 0, 0, 0, 0, 0, 0]
  last_missed_ant : Outport
  spectr_cnt : Outport  Port=2
  recv_errctr : Outport  Port=3
  timeout_errctr : Outport  Port=4
  pktdisc_errctr : Outport  Port=5
  wires:
  Delay1/1(q) -> Register/2, Counter1/1
  Delay3/1(q) -> ant_cnt/2
  Delay2/1(q) -> Counter1/2, ant_cnt/1
  Counter1/1 -> Delay11/1(d)
  Register/1 -> Delay15/1(d)
  ant_cnt/1 -> Slice/1
  Slice/1 -> Register/1
  [reord_timeouterr0] -> Delay97/1(d)
  Logical3/1 -> sync_ctr6/2
  Delay96/1(q) -> sync_ctr1/1, sync_ctr5/1, sync_ctr6/1
  Delay97/1(q) -> Logical3/2
  [cnt_rst] -> Delay96/1(d)
  [reord_valid0] -> Delay98/1(d)
  Delay98/1(q) -> Logical2/1, Logical1/1, Logical3/1
  Logical1/1 -> sync_ctr5/2
  Delay8/1(q) -> Logical1/2
  [reord_pktdisc0] -> Delay8/1(d)
  sync_ctr6/1 -> Delay5/1(d)
  sync_ctr5/1 -> Delay6/1(d)
  sync_ctr1/1 -> Delay4/1(d)
  Delay4/1(q) -> recv_errctr/1
  Delay5/1(q) -> timeout_errctr/1
  Delay6/1(q) -> pktdisc_errctr/1
  Logical2/1 -> sync_ctr1/2
  Delay7/1(q) -> Logical2/2
  [reord_recverr0] -> Delay7/1(d)
  [cnt_rst] -> Delay1/1(d)
  [reord_sync0] -> Delay2/1(d)
  [reord_valid0] -> Delay3/1(d)
  [reord_recverr0] -> Delay9/1(d)
  Delay11/1(q) -> spectr_cnt/1
  Delay15/1(q) -> Convert/1
  Convert/1 -> last_missed_ant/1
  Delay9/1(q) -> Register/3
